simulink model "attitude_ctrl"  (R2026b)
settings: Solver=VariableStepAuto
undefined symbols (not defined in the file): p
settings Model: Creator=lorenzomonti  LastModifiedBy=lorenzomonti

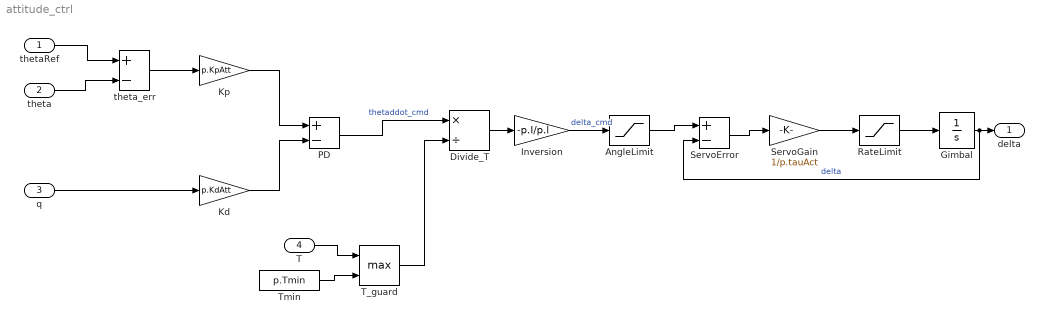
== system attitude_ctrl ==
  thetaRef : Inport
  theta : Inport  Port=2
  q : Inport  Port=3
  T : Inport  Port=4
  AngleLimit : Saturate  UpperLimit=p.deltaMax  LowerLimit=-p.deltaMax
  Divide_T : Product  Inputs=*/
  Gimbal : Integrator
  Inversion : Gain  Gain=-p.I/p.l
  Kd : Gain  Gain=p.KdAtt
  Kp : Gain  Gain=p.KpAtt
  PD : Sum  Inputs=+-
  RateLimit : Saturate  UpperLimit=p.deltaRate  LowerLimit=-p.deltaRate
  ServoError : Sum  Inputs=+-
  ServoGain : Gain  Gain=1/p.tauAct
  T_guard : MinMax  Function=max  Inputs=2
  Tmin : Constant  Value=p.Tmin
  theta_err : Sum  Inputs=+-
  delta : Outport
  wires:
  thetaRef/1 -> theta_err/1
  PD/1 -> Divide_T/1  "thetaddot_cmd"
  theta/1 -> theta_err/2
  Divide_T/1 -> Inversion/1
  Kp/1 -> PD/1
  RateLimit/1 -> Gimbal/1
  T_guard/1 -> Divide_T/2
  Inversion/1 -> AngleLimit/1  "delta_cmd"
  Gimbal/1 -> delta/1, ServoError/2  "delta"
  AngleLimit/1 -> ServoError/1
  Kd/1 -> PD/2
  theta_err/1 -> Kp/1
  Tmin/1 -> T_guard/2
  q/1 -> Kd/1
  T/1 -> T_guard/1
  ServoGain/1 -> RateLimit/1
  ServoError/1 -> ServoGain/1
